simulink model "sim"  (R2025a)
settings: Solver=ode23  StartTime=0.0  StopTime=0.25  RelTol=1e-3
values from neighbouring files (symbols this model uses):
  D = 0.25    [lw6.m]
  i_p = n_nom/n_rpm    (= 14.0622222222)    [lw6.m]
  J_gv = ro_gv*pi*(D/2)^4*h/2    (= 0.0118116520667)    [lw6.m]
  J_sum = 35.9e-7    (= 3.59e-06)    [lw6.m]
  k1 = 0.194    [lw6.m]
  k2 = 0.032    [lw6.m]
  k_m = 19.9e-3    (= 0.0199)    [lw6.m]
  L_a = 0.070e-3    (= 7e-05)    [lw6.m]
  Lxb = 0.19    [lw7.m]
  Lym = 0.31    [lw7.m]
  Lzb = 0.21    [lw7.m]
  R_a = 0.358    [lw6.m]
  ro = 1000    [lw6.m]
  Sat_low = -20    [lw7.m]
  Sat_up = 20    [lw7.m]
  U_nom = 18    [lw6.m]
  w_0 = n_0 * 2 * pi / 60    (= 899.542696478)    [lw6.m]
settings Model: Creator=user  LastModifiedBy=user

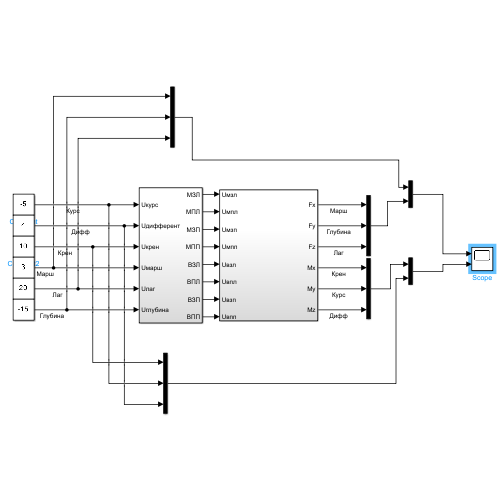
[thumbnail: Simulink's stored preview of the top-level diagram]
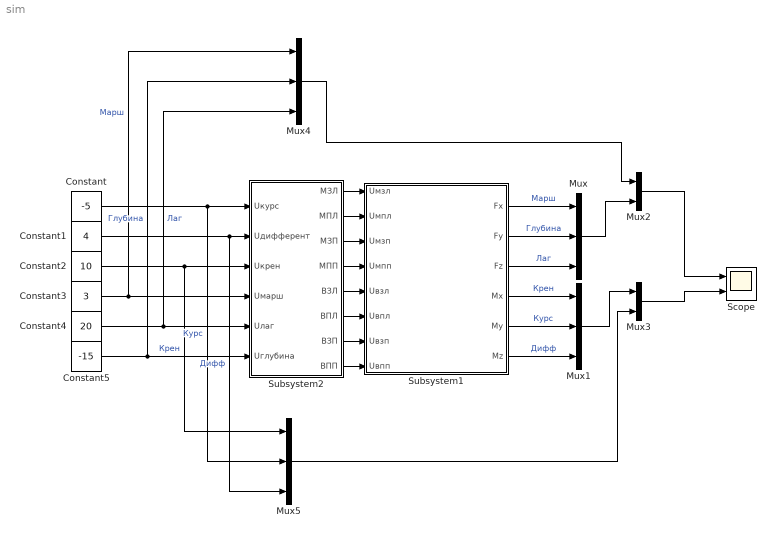
== system sim ==
  Constant : Constant  Value=-5
  Constant1 : Constant  Value=4
  Constant2 : Constant  Value=10
  Constant3 : Constant  Value=3
  Constant4 : Constant  Value=20
  Constant5 : Constant  Value=-15
  Mux{,1,4..5} (4 alike) : Mux  Inputs=3
  Mux2 : Mux  Inputs=2
  Mux3 : Mux  Inputs=2
  Scope : Scope  NumInputPorts=2
      settings: ActiveDisplayYMinimum=-182.36287802568089  ActiveDisplayYMaximum=185.56070658532056
  Subsystem1 : Subsystem
  Subsystem2 : Subsystem
  wires:
  Subsystem1/1(Fx) -> Mux/1  "Марш"
  Subsystem1/3(Fz) -> Mux/3  "Лаг"
  Mux1/1 -> Mux3/1
  Mux/1 -> Mux2/2
  Subsystem1/5(My) -> Mux1/2  "Курс"
  Subsystem1/2(Fy) -> Mux/2  "Глубина"
  Subsystem1/4(Mx) -> Mux1/1  "Крен"
  Subsystem1/6(Mz) -> Mux1/3  "Дифф"
  Subsystem2/1(МЗЛ) -> Subsystem1/1(Uмзл)
  Subsystem2/2(МПЛ) -> Subsystem1/2(Uмпл)
  Subsystem2/3(МЗП) -> Subsystem1/3(Uмзп)
  Subsystem2/4(МПП) -> Subsystem1/4(Uмпп)
  Subsystem2/5(ВЗЛ) -> Subsystem1/5(Uвзл)
  Subsystem2/6(ВПЛ) -> Subsystem1/6(Uвпл)
  Subsystem2/7(ВЗП) -> Subsystem1/7(Uвзп)
  Subsystem2/8(ВПП) -> Subsystem1/8(Uвпп)
  Constant/1 -> Mux5/2, Subsystem2/1(Uкурс)  "Курс"
  Constant1/1 -> Mux5/3, Subsystem2/2(Uдифферент)  "Дифф"
  Constant2/1 -> Subsystem2/3(Uкрен), Mux5/1  "Крен"
  Constant3/1 -> Subsystem2/4(Uмарш), Mux4/1  "Марш"
  Constant4/1 -> Subsystem2/5(Uлаг), Mux4/3  "Лаг"
  Constant5/1 -> Subsystem2/6(Uглубина), Mux4/2  "Глубина"
  Mux2/1 -> Scope/1
  Mux3/1 -> Scope/2
  Mux4/1 -> Mux2/1
  Mux5/1 -> Mux3/2

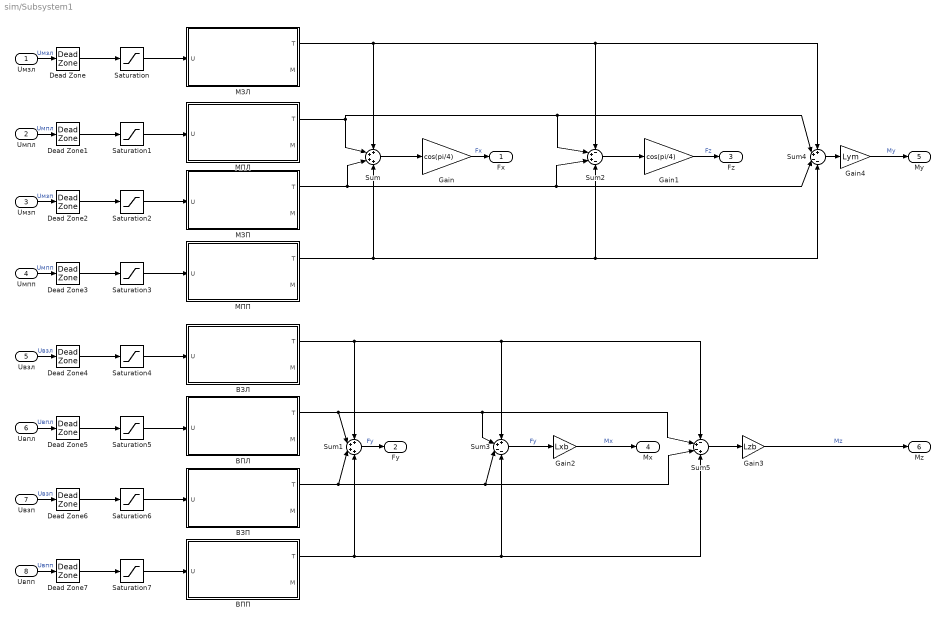
== system sim/Subsystem1 ==
  Uмзл : Inport
  Uмпл : Inport  Port=2
  Uмзп : Inport  Port=3
  Uмпп : Inport  Port=4
  Uвзл : Inport  Port=5
  Uвпл : Inport  Port=6
  Uвзп : Inport  Port=7
  Uвпп : Inport  Port=8
  Dead Zone{,1..7} (8 alike) : DeadZone  LowerValue=Dead_low  UpperValue=Dead_up
  Gain : Gain  Gain=cos(pi/4)
  Gain1 : Gain  Gain=cos(pi/4)
  Gain2 : Gain  Gain=Lxb
  Gain3 : Gain  Gain=Lzb
  Gain4 : Gain  Gain=Lym
  Saturation{,1..7} (8 alike) : Saturate  UpperLimit=Sat_up  LowerLimit=Sat_low
  Sum : Sum  Inputs=++++
  Sum1 : Sum  Inputs=++++
  Sum2 : Sum  Inputs=-++-
  Sum3 : Sum  Inputs=++--
  Sum4 : Sum  Inputs=++--
  Sum5 : Sum  Inputs=-+-+
  ВЗЛ : Subsystem
  ВЗП : Subsystem
  ВПЛ : Subsystem
  ВПП : Subsystem
  МЗЛ : Subsystem
  МЗП : Subsystem
  МПЛ : Subsystem
  МПП : Subsystem
  Fx : Outport
  Fy : Outport  Port=2
  Fz : Outport  Port=3
  Mx : Outport  Port=4
  My : Outport  Port=5
  Mz : Outport  Port=6
  wires:
  Uвзл/1 -> Dead Zone4/1  "Uвзл"
  Sum4/1 -> Gain4/1
  Gain1/1 -> Fz/1  "Fz"
  Sum5/1 -> Gain3/1
  Uвпл/1 -> Dead Zone5/1  "Uвпл"
  Gain/1 -> Fx/1  "Fx"
  Sum/1 -> Gain/1
  Sum1/1 -> Fy/1  "Fy"
  Gain4/1 -> My/1  "My"
  ВЗП/1(T) -> Sum5/3, Sum3/3, Sum1/3
  Uмпп/1 -> Dead Zone3/1  "Uмпп"
  Sum3/1 -> Gain2/1  "Fy"
  Uвпп/1 -> Dead Zone7/1  "Uвпп"
  Sum2/1 -> Gain1/1
  МЗЛ/1(T) -> Sum4/1, Sum2/1, Sum/1
  ВПЛ/1(T) -> Sum5/2, Sum3/2, Sum1/2
  Uмпл/1 -> Dead Zone1/1  "Uмпл"
  Uмзл/1 -> Dead Zone/1  "Uмзл"
  Uвзп/1 -> Dead Zone6/1  "Uвзп"
  Dead Zone3/1 -> Saturation3/1
  МЗП/1(T) -> Sum4/3, Sum2/3, Sum/3
  МПЛ/1(T) -> Sum4/2, Sum2/2, Sum/2
  МПП/1(T) -> Sum4/4, Sum2/4, Sum/4
  Saturation7/1 -> ВПП/1(U)
  Saturation3/1 -> МПП/1(U)
  Saturation6/1 -> ВЗП/1(U)
  Saturation2/1 -> МЗП/1(U)
  Dead Zone1/1 -> Saturation1/1
  Dead Zone2/1 -> Saturation2/1
  Uмзп/1 -> Dead Zone2/1  "Uмзп"
  ВПП/1(T) -> Sum5/4, Sum3/4, Sum1/4
  Saturation/1 -> МЗЛ/1(U)
  Gain3/1 -> Mz/1  "Mz"
  Saturation5/1 -> ВПЛ/1(U)
  ВЗЛ/1(T) -> Sum5/1, Sum3/1, Sum1/1
  Dead Zone7/1 -> Saturation7/1
  Dead Zone4/1 -> Saturation4/1
  Gain2/1 -> Mx/1  "Mx"
  Dead Zone5/1 -> Saturation5/1
  Dead Zone/1 -> Saturation/1
  Dead Zone6/1 -> Saturation6/1
  Saturation4/1 -> ВЗЛ/1(U)
  Saturation1/1 -> МПЛ/1(U)

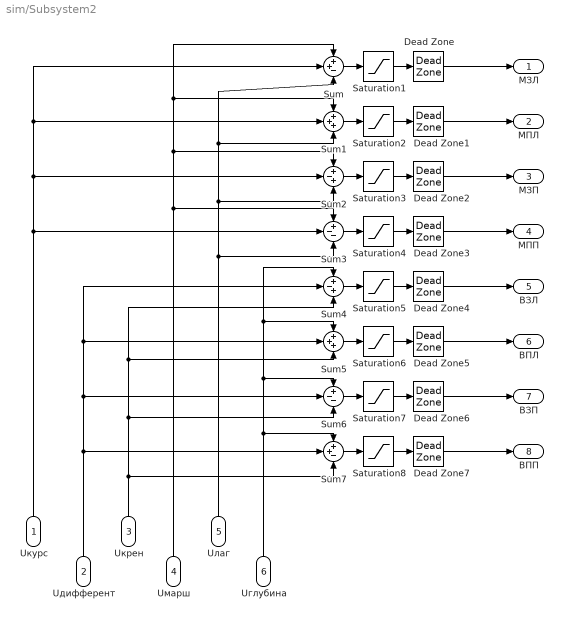
== system sim/Subsystem2 ==
  Uкурс : Inport
  Uдифферент : Inport  Port=2
  Uкрен : Inport  Port=3
  Uмарш : Inport  Port=4
  Uлаг : Inport  Port=5
  Uглубина : Inport  Port=6
  Dead Zone{,1..7} (8 alike) : DeadZone  LowerValue=Dead_low  UpperValue=Dead_up
  Saturation{1..8} (8 alike) : Saturate  UpperLimit=Sat_up  LowerLimit=Sat_low
  Sum : Sum  Inputs=++-
  Sum1 : Sum  Inputs=+++
  Sum2 : Sum  Inputs=+-+
  Sum3 : Sum  Inputs=+--
  Sum4 : Sum  Inputs=+-+
  Sum5 : Sum  Inputs=+++
  Sum6 : Sum  Inputs=+--
  Sum7 : Sum  Inputs=++-
  МЗЛ : Outport
  МПЛ : Outport  Port=2
  МЗП : Outport  Port=3
  МПП : Outport  Port=4
  ВЗЛ : Outport  Port=5
  ВПЛ : Outport  Port=6
  ВЗП : Outport  Port=7
  ВПП : Outport  Port=8
  wires:
  Sum/1 -> Saturation1/1
  Saturation1/1 -> Dead Zone/1
  Dead Zone/1 -> МЗЛ/1
  Sum1/1 -> Saturation2/1
  Saturation2/1 -> Dead Zone1/1
  Dead Zone1/1 -> МПЛ/1
  Sum2/1 -> Saturation3/1
  Saturation3/1 -> Dead Zone2/1
  Dead Zone2/1 -> МЗП/1
  Sum3/1 -> Saturation4/1
  Saturation4/1 -> Dead Zone3/1
  Dead Zone3/1 -> МПП/1
  Sum4/1 -> Saturation5/1
  Sum7/1 -> Saturation8/1
  Saturation8/1 -> Dead Zone7/1
  Saturation5/1 -> Dead Zone4/1
  Saturation6/1 -> Dead Zone5/1
  Sum5/1 -> Saturation6/1
  Saturation7/1 -> Dead Zone6/1
  Sum6/1 -> Saturation7/1
  Dead Zone4/1 -> ВЗЛ/1
  Dead Zone5/1 -> ВПЛ/1
  Dead Zone6/1 -> ВЗП/1
  Dead Zone7/1 -> ВПП/1
  Uкурс/1 -> Sum3/2, Sum2/2, Sum1/2, Sum/2
  Uдифферент/1 -> Sum7/2, Sum6/2, Sum5/2, Sum4/2
  Uкрен/1 -> Sum7/3, Sum6/3, Sum5/3, Sum4/3
  Uмарш/1 -> Sum3/1, Sum2/1, Sum1/1, Sum/1
  Uлаг/1 -> Sum3/3, Sum2/3, Sum/3, Sum1/3
  Uглубина/1 -> Sum6/1, Sum5/1, Sum4/1, Sum7/1

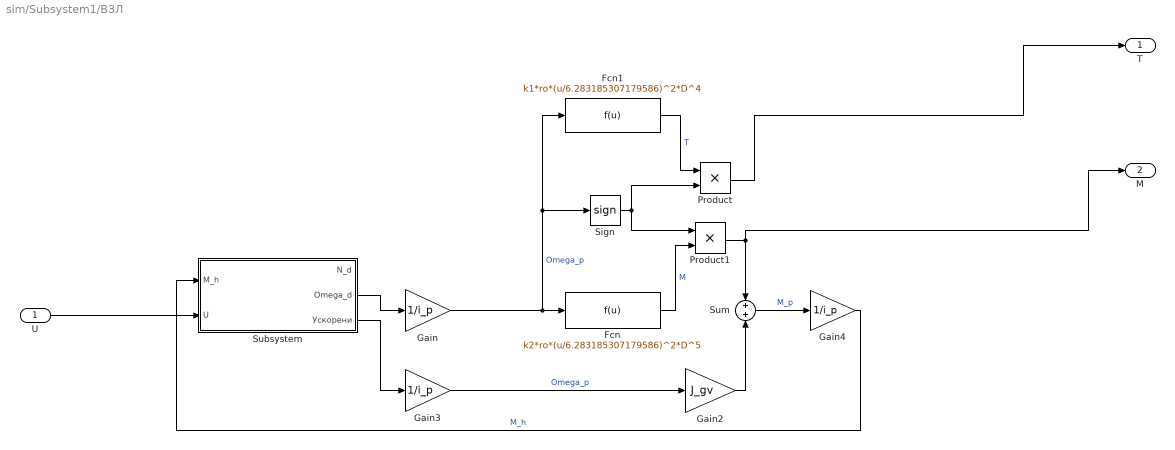
== system sim/Subsystem1/ВЗЛ ==
  U : Inport
  Fcn : Fcn  Expr=k2*ro*(u/6.283185307179586)^2*D^5
  Fcn1 : Fcn  Expr=k1*ro*(u/6.283185307179586)^2*D^4
  Gain : Gain  Gain=1/i_p
  Gain2 : Gain  Gain=J_gv
  Gain3 : Gain  Gain=1/i_p
  Gain4 : Gain  Gain=1/i_p
  Product : Product
  Product1 : Product
  Sign : Signum
  Subsystem : Subsystem
  Sum : Sum
  T : Outport
  M : Outport  Port=2
  wires:
  Gain3/1 -> Gain2/1  "Omega_p"
  Subsystem/3(Ускорени) -> Gain3/1
  Fcn1/1 -> Product/1  "T"
  Subsystem/2(Omega_d) -> Gain/1
  Gain/1 -> Fcn/1, Fcn1/1, Sign/1  "Omega_p"
  Sum/1 -> Gain4/1  "M_p"
  Sign/1 -> Product/2, Product1/1
  Product/1 -> T/1
  Gain4/1 -> Subsystem/1(M_h)  "M_h"
  Product1/1 -> Sum/1, M/1
  U/1 -> Subsystem/2(U)
  Fcn/1 -> Product1/2  "M"
  Gain2/1 -> Sum/2

== system sim/Subsystem1/ВЗП ==
  U : Inport
  Fcn : Fcn  Expr=k2*ro*(u/6.283185307179586)^2*D^5
  Fcn1 : Fcn  Expr=k1*ro*(u/6.283185307179586)^2*D^4
  Gain : Gain  Gain=1/i_p
  Gain2 : Gain  Gain=J_gv
  Gain3 : Gain  Gain=1/i_p
  Gain4 : Gain  Gain=1/i_p
  Product : Product
  Product1 : Product
  Sign : Signum
  Subsystem : Subsystem
  Sum : Sum
  T : Outport
  M : Outport  Port=2
  wires:
  Gain3/1 -> Gain2/1  "Omega_p"
  Subsystem/3(Ускорени) -> Gain3/1
  Fcn1/1 -> Product/1  "T"
  Subsystem/2(Omega_d) -> Gain/1
  Gain/1 -> Fcn/1, Fcn1/1, Sign/1  "Omega_p"
  Sum/1 -> Gain4/1  "M_p"
  Sign/1 -> Product/2, Product1/1
  Product/1 -> T/1
  Gain4/1 -> Subsystem/1(M_h)  "M_h"
  Product1/1 -> Sum/1, M/1
  U/1 -> Subsystem/2(U)
  Fcn/1 -> Product1/2  "M"
  Gain2/1 -> Sum/2

== system sim/Subsystem1/ВПЛ ==
  U : Inport
  Fcn : Fcn  Expr=k2*ro*(u/6.283185307179586)^2*D^5
  Fcn1 : Fcn  Expr=k1*ro*(u/6.283185307179586)^2*D^4
  Gain : Gain  Gain=1/i_p
  Gain2 : Gain  Gain=J_gv
  Gain3 : Gain  Gain=1/i_p
  Gain4 : Gain  Gain=1/i_p
  Product : Product
  Product1 : Product
  Sign : Signum
  Subsystem : Subsystem
  Sum : Sum
  T : Outport
  M : Outport  Port=2
  wires:
  Gain3/1 -> Gain2/1  "Omega_p"
  Subsystem/3(Ускорени) -> Gain3/1
  Fcn1/1 -> Product/1  "T"
  Subsystem/2(Omega_d) -> Gain/1
  Gain/1 -> Fcn/1, Fcn1/1, Sign/1  "Omega_p"
  Sum/1 -> Gain4/1  "M_p"
  Sign/1 -> Product/2, Product1/1
  Product/1 -> T/1
  Gain4/1 -> Subsystem/1(M_h)  "M_h"
  Product1/1 -> Sum/1, M/1
  U/1 -> Subsystem/2(U)
  Fcn/1 -> Product1/2  "M"
  Gain2/1 -> Sum/2

== system sim/Subsystem1/ВПП ==
  U : Inport
  Fcn : Fcn  Expr=k2*ro*(u/6.283185307179586)^2*D^5
  Fcn1 : Fcn  Expr=k1*ro*(u/6.283185307179586)^2*D^4
  Gain : Gain  Gain=1/i_p
  Gain2 : Gain  Gain=J_gv
  Gain3 : Gain  Gain=1/i_p
  Gain4 : Gain  Gain=1/i_p
  Product : Product
  Product1 : Product
  Sign : Signum
  Subsystem : Subsystem
  Sum : Sum
  T : Outport
  M : Outport  Port=2
  wires:
  Gain3/1 -> Gain2/1  "Omega_p"
  Subsystem/3(Ускорени) -> Gain3/1
  Fcn1/1 -> Product/1  "T"
  Subsystem/2(Omega_d) -> Gain/1
  Gain/1 -> Fcn/1, Fcn1/1, Sign/1  "Omega_p"
  Sum/1 -> Gain4/1  "M_p"
  Sign/1 -> Product/2, Product1/1
  Product/1 -> T/1
  Gain4/1 -> Subsystem/1(M_h)  "M_h"
  Product1/1 -> Sum/1, M/1
  U/1 -> Subsystem/2(U)
  Fcn/1 -> Product1/2  "M"
  Gain2/1 -> Sum/2

== system sim/Subsystem1/МЗЛ ==
  U : Inport
  Fcn : Fcn  Expr=k2*ro*(u/6.283185307179586)^2*D^5
  Fcn1 : Fcn  Expr=k1*ro*(u/6.283185307179586)^2*D^4
  Gain : Gain  Gain=1/i_p
  Gain2 : Gain  Gain=J_gv
  Gain3 : Gain  Gain=1/i_p
  Gain4 : Gain  Gain=1/i_p
  Product : Product
  Product1 : Product
  Sign : Signum
  Subsystem : Subsystem
  Sum : Sum
  T : Outport
  M : Outport  Port=2
  wires:
  Gain3/1 -> Gain2/1  "Omega_p"
  Subsystem/3(Ускорени) -> Gain3/1
  Fcn1/1 -> Product/1  "T"
  Subsystem/2(Omega_d) -> Gain/1
  Gain/1 -> Fcn/1, Fcn1/1, Sign/1  "Omega_p"
  Sum/1 -> Gain4/1  "M_p"
  Sign/1 -> Product/2, Product1/1
  Product/1 -> T/1
  Gain4/1 -> Subsystem/1(M_h)  "M_h"
  Product1/1 -> Sum/1, M/1
  U/1 -> Subsystem/2(U)
  Fcn/1 -> Product1/2  "M"
  Gain2/1 -> Sum/2

== system sim/Subsystem1/МЗП ==
  U : Inport
  Fcn : Fcn  Expr=k2*ro*(u/6.283185307179586)^2*D^5
  Fcn1 : Fcn  Expr=k1*ro*(u/6.283185307179586)^2*D^4
  Gain : Gain  Gain=1/i_p
  Gain2 : Gain  Gain=J_gv
  Gain3 : Gain  Gain=1/i_p
  Gain4 : Gain  Gain=1/i_p
  Product : Product
  Product1 : Product
  Sign : Signum
  Subsystem : Subsystem
  Sum : Sum
  T : Outport
  M : Outport  Port=2
  wires:
  Gain3/1 -> Gain2/1  "Omega_p"
  Subsystem/3(Ускорени) -> Gain3/1
  Fcn1/1 -> Product/1  "T"
  Subsystem/2(Omega_d) -> Gain/1
  Gain/1 -> Fcn/1, Fcn1/1, Sign/1  "Omega_p"
  Sum/1 -> Gain4/1  "M_p"
  Sign/1 -> Product/2, Product1/1
  Product/1 -> T/1
  Gain4/1 -> Subsystem/1(M_h)  "M_h"
  Product1/1 -> Sum/1, M/1
  U/1 -> Subsystem/2(U)
  Fcn/1 -> Product1/2  "M"
  Gain2/1 -> Sum/2

== system sim/Subsystem1/МПЛ ==
  U : Inport
  Fcn : Fcn  Expr=k2*ro*(u/6.283185307179586)^2*D^5
  Fcn1 : Fcn  Expr=k1*ro*(u/6.283185307179586)^2*D^4
  Gain : Gain  Gain=1/i_p
  Gain2 : Gain  Gain=J_gv
  Gain3 : Gain  Gain=1/i_p
  Gain4 : Gain  Gain=1/i_p
  Product : Product
  Product1 : Product
  Sign : Signum
  Subsystem : Subsystem
  Sum : Sum
  T : Outport
  M : Outport  Port=2
  wires:
  Gain3/1 -> Gain2/1  "Omega_p"
  Subsystem/3(Ускорени) -> Gain3/1
  Fcn1/1 -> Product/1  "T"
  Subsystem/2(Omega_d) -> Gain/1
  Gain/1 -> Fcn/1, Fcn1/1, Sign/1  "Omega_p"
  Sum/1 -> Gain4/1  "M_p"
  Sign/1 -> Product/2, Product1/1
  Product/1 -> T/1
  Gain4/1 -> Subsystem/1(M_h)  "M_h"
  Product1/1 -> Sum/1, M/1
  U/1 -> Subsystem/2(U)
  Fcn/1 -> Product1/2  "M"
  Gain2/1 -> Sum/2

== system sim/Subsystem1/МПП ==
  U : Inport
  Fcn : Fcn  Expr=k2*ro*(u/6.283185307179586)^2*D^5
  Fcn1 : Fcn  Expr=k1*ro*(u/6.283185307179586)^2*D^4
  Gain : Gain  Gain=1/i_p
  Gain2 : Gain  Gain=J_gv
  Gain3 : Gain  Gain=1/i_p
  Gain4 : Gain  Gain=1/i_p
  Product : Product
  Product1 : Product
  Sign : Signum
  Subsystem : Subsystem
  Sum : Sum
  T : Outport
  M : Outport  Port=2
  wires:
  Gain3/1 -> Gain2/1  "Omega_p"
  Subsystem/3(Ускорени) -> Gain3/1
  Fcn1/1 -> Product/1  "T"
  Subsystem/2(Omega_d) -> Gain/1
  Gain/1 -> Fcn/1, Fcn1/1, Sign/1  "Omega_p"
  Sum/1 -> Gain4/1  "M_p"
  Sign/1 -> Product/2, Product1/1
  Product/1 -> T/1
  Gain4/1 -> Subsystem/1(M_h)  "M_h"
  Product1/1 -> Sum/1, M/1
  U/1 -> Subsystem/2(U)
  Fcn/1 -> Product1/2  "M"
  Gain2/1 -> Sum/2

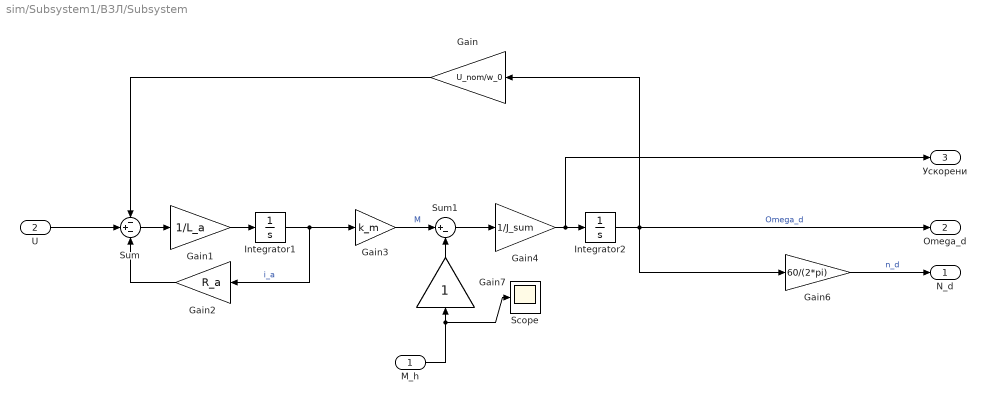
== system sim/Subsystem1/ВЗЛ/Subsystem ==
  M_h : Inport
  U : Inport  Port=2
  Gain : Gain  Gain=U_nom/w_0
  Gain1 : Gain  Gain=1/L_a
  Gain2 : Gain  Gain=R_a
  Gain3 : Gain  Gain=k_m
  Gain4 : Gain  Gain=1/J_sum
  Gain6 : Gain  Gain=60/(2*pi)
  Gain7 : Gain
  Integrator1 : Integrator
  Integrator2 : Integrator
  Scope : Scope
      settings: ActiveDisplayYMinimum=-1  ActiveDisplayYMaximum=1
  Sum : Sum  Inputs=-+-
  Sum1 : Sum  Inputs=|+-
  N_d : Outport
  Omega_d : Outport  Port=2
  Ускорени : Outport  Port=3
  wires:
  U/1 -> Sum/2
  Gain3/1 -> Sum1/1  "M"
  M_h/1 -> Scope/1, Gain7/1
  Gain6/1 -> N_d/1  "n_d"
  Gain1/1 -> Integrator1/1
  Integrator1/1 -> Gain3/1, Gain2/1  "i_a"
  Integrator2/1 -> Omega_d/1, Gain6/1, Gain/1  "Omega_d"
  Gain4/1 -> Ускорени/1, Integrator2/1
  Sum/1 -> Gain1/1
  Gain2/1 -> Sum/3
  Gain7/1 -> Sum1/2
  Gain/1 -> Sum/1
  Sum1/1 -> Gain4/1

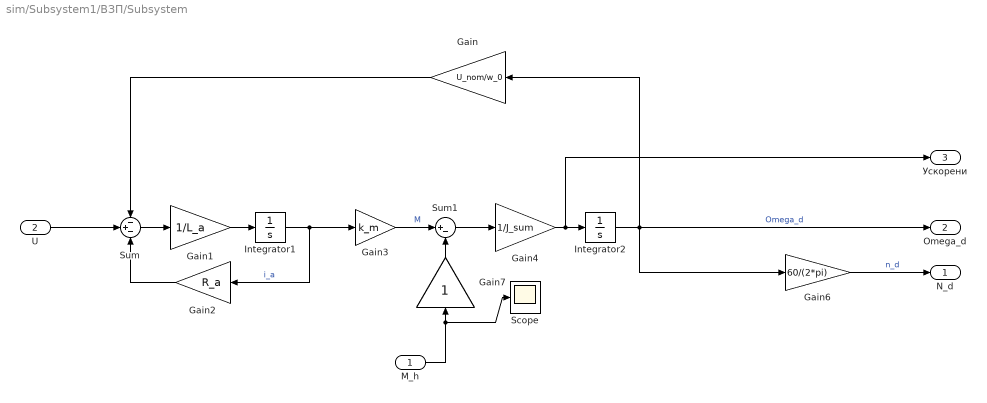
== system sim/Subsystem1/ВЗП/Subsystem ==
  M_h : Inport
  U : Inport  Port=2
  Gain : Gain  Gain=U_nom/w_0
  Gain1 : Gain  Gain=1/L_a
  Gain2 : Gain  Gain=R_a
  Gain3 : Gain  Gain=k_m
  Gain4 : Gain  Gain=1/J_sum
  Gain6 : Gain  Gain=60/(2*pi)
  Gain7 : Gain
  Integrator1 : Integrator
  Integrator2 : Integrator
  Scope : Scope
      settings: ActiveDisplayYMinimum=-1  ActiveDisplayYMaximum=1
  Sum : Sum  Inputs=-+-
  Sum1 : Sum  Inputs=|+-
  N_d : Outport
  Omega_d : Outport  Port=2
  Ускорени : Outport  Port=3
  wires:
  U/1 -> Sum/2
  Gain3/1 -> Sum1/1  "M"
  M_h/1 -> Scope/1, Gain7/1
  Gain6/1 -> N_d/1  "n_d"
  Gain1/1 -> Integrator1/1
  Integrator1/1 -> Gain3/1, Gain2/1  "i_a"
  Integrator2/1 -> Omega_d/1, Gain6/1, Gain/1  "Omega_d"
  Gain4/1 -> Ускорени/1, Integrator2/1
  Sum/1 -> Gain1/1
  Gain2/1 -> Sum/3
  Gain7/1 -> Sum1/2
  Gain/1 -> Sum/1
  Sum1/1 -> Gain4/1

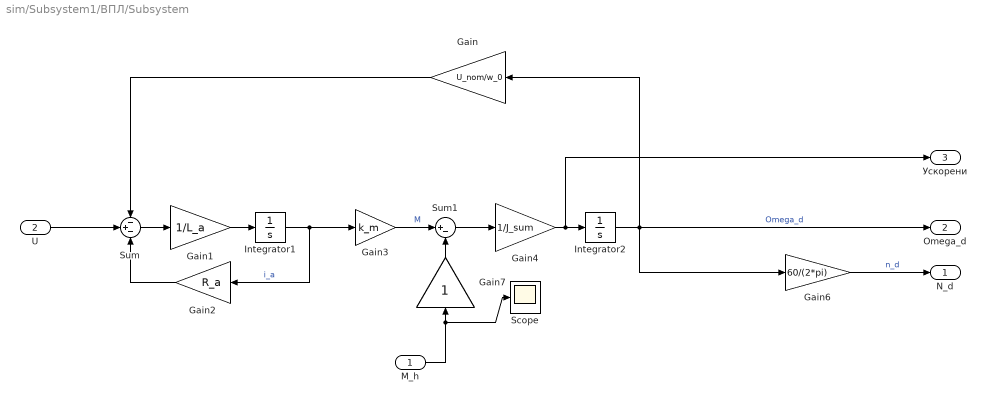
== system sim/Subsystem1/ВПЛ/Subsystem ==
  M_h : Inport
  U : Inport  Port=2
  Gain : Gain  Gain=U_nom/w_0
  Gain1 : Gain  Gain=1/L_a
  Gain2 : Gain  Gain=R_a
  Gain3 : Gain  Gain=k_m
  Gain4 : Gain  Gain=1/J_sum
  Gain6 : Gain  Gain=60/(2*pi)
  Gain7 : Gain
  Integrator1 : Integrator
  Integrator2 : Integrator
  Scope : Scope
      settings: ActiveDisplayYMinimum=-1  ActiveDisplayYMaximum=1
  Sum : Sum  Inputs=-+-
  Sum1 : Sum  Inputs=|+-
  N_d : Outport
  Omega_d : Outport  Port=2
  Ускорени : Outport  Port=3
  wires:
  U/1 -> Sum/2
  Gain3/1 -> Sum1/1  "M"
  M_h/1 -> Scope/1, Gain7/1
  Gain6/1 -> N_d/1  "n_d"
  Gain1/1 -> Integrator1/1
  Integrator1/1 -> Gain3/1, Gain2/1  "i_a"
  Integrator2/1 -> Omega_d/1, Gain6/1, Gain/1  "Omega_d"
  Gain4/1 -> Ускорени/1, Integrator2/1
  Sum/1 -> Gain1/1
  Gain2/1 -> Sum/3
  Gain7/1 -> Sum1/2
  Gain/1 -> Sum/1
  Sum1/1 -> Gain4/1

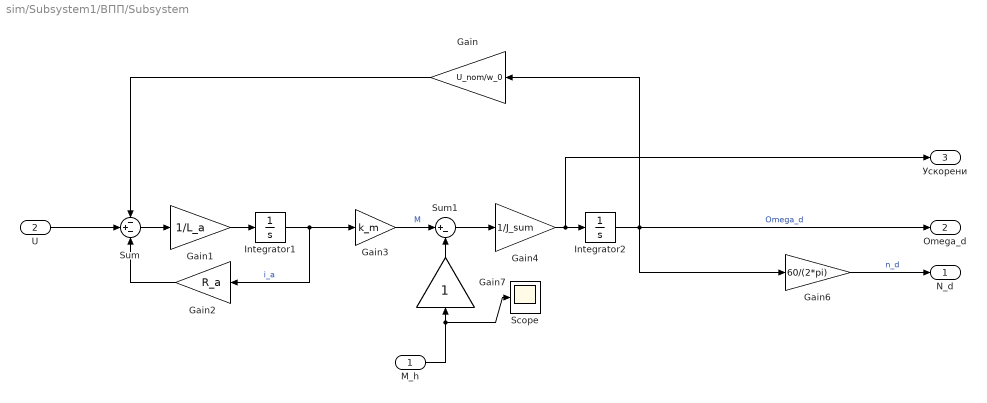
== system sim/Subsystem1/ВПП/Subsystem ==
  M_h : Inport
  U : Inport  Port=2
  Gain : Gain  Gain=U_nom/w_0
  Gain1 : Gain  Gain=1/L_a
  Gain2 : Gain  Gain=R_a
  Gain3 : Gain  Gain=k_m
  Gain4 : Gain  Gain=1/J_sum
  Gain6 : Gain  Gain=60/(2*pi)
  Gain7 : Gain
  Integrator1 : Integrator
  Integrator2 : Integrator
  Scope : Scope
      settings: ActiveDisplayYMinimum=-1  ActiveDisplayYMaximum=1
  Sum : Sum  Inputs=-+-
  Sum1 : Sum  Inputs=|+-
  N_d : Outport
  Omega_d : Outport  Port=2
  Ускорени : Outport  Port=3
  wires:
  U/1 -> Sum/2
  Gain3/1 -> Sum1/1  "M"
  M_h/1 -> Scope/1, Gain7/1
  Gain6/1 -> N_d/1  "n_d"
  Gain1/1 -> Integrator1/1
  Integrator1/1 -> Gain3/1, Gain2/1  "i_a"
  Integrator2/1 -> Omega_d/1, Gain6/1, Gain/1  "Omega_d"
  Gain4/1 -> Ускорени/1, Integrator2/1
  Sum/1 -> Gain1/1
  Gain2/1 -> Sum/3
  Gain7/1 -> Sum1/2
  Gain/1 -> Sum/1
  Sum1/1 -> Gain4/1

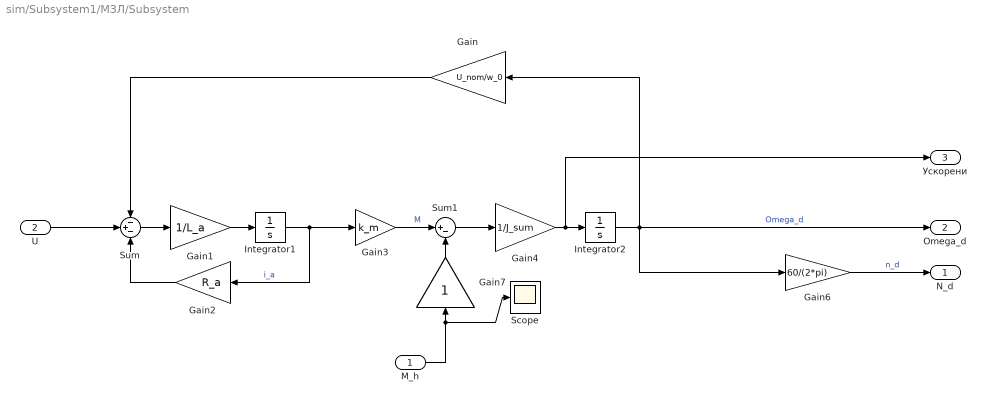
== system sim/Subsystem1/МЗЛ/Subsystem ==
  M_h : Inport
  U : Inport  Port=2
  Gain : Gain  Gain=U_nom/w_0
  Gain1 : Gain  Gain=1/L_a
  Gain2 : Gain  Gain=R_a
  Gain3 : Gain  Gain=k_m
  Gain4 : Gain  Gain=1/J_sum
  Gain6 : Gain  Gain=60/(2*pi)
  Gain7 : Gain
  Integrator1 : Integrator
  Integrator2 : Integrator
  Scope : Scope
      settings: ActiveDisplayYMinimum=-1  ActiveDisplayYMaximum=1
  Sum : Sum  Inputs=-+-
  Sum1 : Sum  Inputs=|+-
  N_d : Outport
  Omega_d : Outport  Port=2
  Ускорени : Outport  Port=3
  wires:
  U/1 -> Sum/2
  Gain3/1 -> Sum1/1  "M"
  M_h/1 -> Scope/1, Gain7/1
  Gain6/1 -> N_d/1  "n_d"
  Gain1/1 -> Integrator1/1
  Integrator1/1 -> Gain3/1, Gain2/1  "i_a"
  Integrator2/1 -> Omega_d/1, Gain6/1, Gain/1  "Omega_d"
  Gain4/1 -> Ускорени/1, Integrator2/1
  Sum/1 -> Gain1/1
  Gain2/1 -> Sum/3
  Gain7/1 -> Sum1/2
  Gain/1 -> Sum/1
  Sum1/1 -> Gain4/1

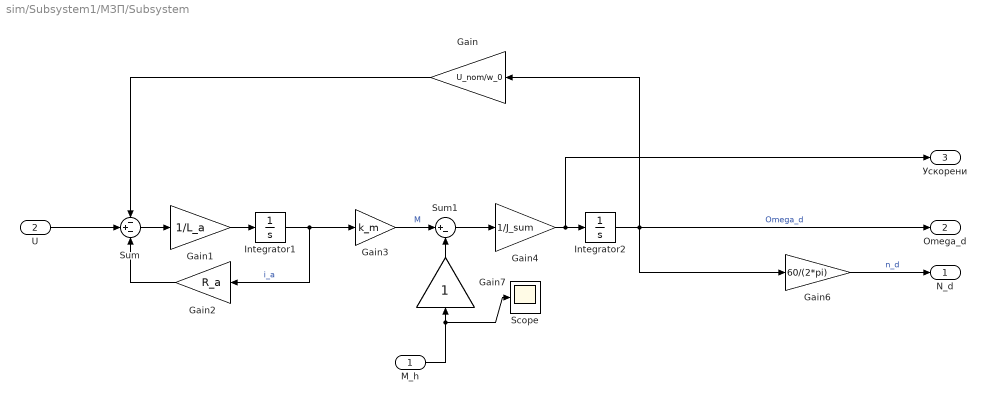
== system sim/Subsystem1/МЗП/Subsystem ==
  M_h : Inport
  U : Inport  Port=2
  Gain : Gain  Gain=U_nom/w_0
  Gain1 : Gain  Gain=1/L_a
  Gain2 : Gain  Gain=R_a
  Gain3 : Gain  Gain=k_m
  Gain4 : Gain  Gain=1/J_sum
  Gain6 : Gain  Gain=60/(2*pi)
  Gain7 : Gain
  Integrator1 : Integrator
  Integrator2 : Integrator
  Scope : Scope
      settings: ActiveDisplayYMinimum=-1  ActiveDisplayYMaximum=1
  Sum : Sum  Inputs=-+-
  Sum1 : Sum  Inputs=|+-
  N_d : Outport
  Omega_d : Outport  Port=2
  Ускорени : Outport  Port=3
  wires:
  U/1 -> Sum/2
  Gain3/1 -> Sum1/1  "M"
  M_h/1 -> Scope/1, Gain7/1
  Gain6/1 -> N_d/1  "n_d"
  Gain1/1 -> Integrator1/1
  Integrator1/1 -> Gain3/1, Gain2/1  "i_a"
  Integrator2/1 -> Omega_d/1, Gain6/1, Gain/1  "Omega_d"
  Gain4/1 -> Ускорени/1, Integrator2/1
  Sum/1 -> Gain1/1
  Gain2/1 -> Sum/3
  Gain7/1 -> Sum1/2
  Gain/1 -> Sum/1
  Sum1/1 -> Gain4/1

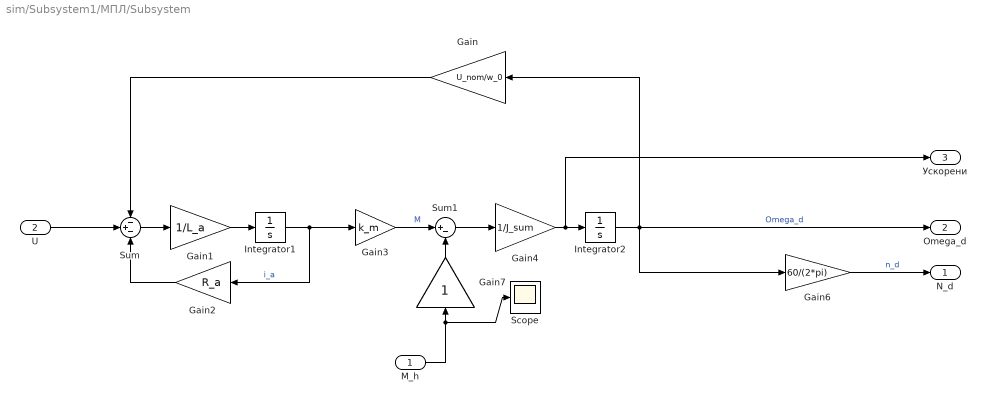
== system sim/Subsystem1/МПЛ/Subsystem ==
  M_h : Inport
  U : Inport  Port=2
  Gain : Gain  Gain=U_nom/w_0
  Gain1 : Gain  Gain=1/L_a
  Gain2 : Gain  Gain=R_a
  Gain3 : Gain  Gain=k_m
  Gain4 : Gain  Gain=1/J_sum
  Gain6 : Gain  Gain=60/(2*pi)
  Gain7 : Gain
  Integrator1 : Integrator
  Integrator2 : Integrator
  Scope : Scope
      settings: ActiveDisplayYMinimum=-1  ActiveDisplayYMaximum=1
  Sum : Sum  Inputs=-+-
  Sum1 : Sum  Inputs=|+-
  N_d : Outport
  Omega_d : Outport  Port=2
  Ускорени : Outport  Port=3
  wires:
  U/1 -> Sum/2
  Gain3/1 -> Sum1/1  "M"
  M_h/1 -> Scope/1, Gain7/1
  Gain6/1 -> N_d/1  "n_d"
  Gain1/1 -> Integrator1/1
  Integrator1/1 -> Gain3/1, Gain2/1  "i_a"
  Integrator2/1 -> Omega_d/1, Gain6/1, Gain/1  "Omega_d"
  Gain4/1 -> Ускорени/1, Integrator2/1
  Sum/1 -> Gain1/1
  Gain2/1 -> Sum/3
  Gain7/1 -> Sum1/2
  Gain/1 -> Sum/1
  Sum1/1 -> Gain4/1

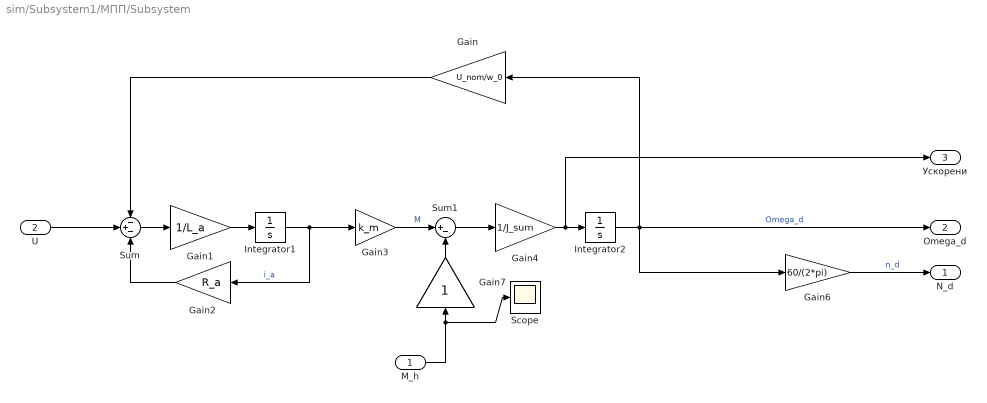
== system sim/Subsystem1/МПП/Subsystem ==
  M_h : Inport
  U : Inport  Port=2
  Gain : Gain  Gain=U_nom/w_0
  Gain1 : Gain  Gain=1/L_a
  Gain2 : Gain  Gain=R_a
  Gain3 : Gain  Gain=k_m
  Gain4 : Gain  Gain=1/J_sum
  Gain6 : Gain  Gain=60/(2*pi)
  Gain7 : Gain
  Integrator1 : Integrator
  Integrator2 : Integrator
  Scope : Scope
      settings: ActiveDisplayYMinimum=-1  ActiveDisplayYMaximum=1
  Sum : Sum  Inputs=-+-
  Sum1 : Sum  Inputs=|+-
  N_d : Outport
  Omega_d : Outport  Port=2
  Ускорени : Outport  Port=3
  wires:
  U/1 -> Sum/2
  Gain3/1 -> Sum1/1  "M"
  M_h/1 -> Scope/1, Gain7/1
  Gain6/1 -> N_d/1  "n_d"
  Gain1/1 -> Integrator1/1
  Integrator1/1 -> Gain3/1, Gain2/1  "i_a"
  Integrator2/1 -> Omega_d/1, Gain6/1, Gain/1  "Omega_d"
  Gain4/1 -> Ускорени/1, Integrator2/1
  Sum/1 -> Gain1/1
  Gain2/1 -> Sum/3
  Gain7/1 -> Sum1/2
  Gain/1 -> Sum/1
  Sum1/1 -> Gain4/1
